simulink model "s_c_nbe_m1k"  (R2016b)
(part 4 of 198)

  [ct_sync] -> Subsystem10/5(in3)
  bus_create2/1(bus_out) -> [tvgtone_level0]
  bus_create3/1(bus_out) -> [tvgtone_level1]
  tvg_tone_levels/2(in_p0i) -> bus_create2/2(in2)
  tvg_tone_levels/3(in_p1r) -> bus_create3/1(in1)
  tvg_tone_levels/4(in_p1i) -> bus_create3/2(in2)
  tvg_tone_levels/1(in_p0r) -> bus_create2/1(in1)
  tvg_tone_targets/1(in_p0) -> Slice18/1
  tvg_tone_targets/2(in_p1) -> Slice19/1
  Constant51/1 -> tvg_tone_targets/1(sim_1)
  Constant52/1 -> tvg_tone_targets/2(sim_2)
  Constant37/1 -> tvg_tone_levels/4(sim_4)
  Constant2/1 -> tvg_tone_levels/1(sim_1)
  Constant27/1 -> tvg_tone_levels/3(sim_3)
  Constant5/1 -> tvg_tone_levels/2(sim_2)
  we_delay49/1(q) -> [ct_tag_insert_sel]
  edge_detect3/1 -> [ct_rst_err_latch]
  we_delay47/1(q) -> edge_detect3/1
  we_delay48/1(q) -> [ct_fake_data_error]
  we_delay13/1(q) -> [ct_tvg_en]
  we_delay50/1(q) -> [ct_tvg_en2]
  Constant7/1 -> ct_control0/5(sim_5)
  Constant21/1 -> ct_control0/4(sim_4)
  Constant20/1 -> ct_control0/3(sim_3)
  Constant22/1 -> ct_control0/2(sim_2)
  Constant15/1 -> ct_control0/1(sim_1)
  ct_control0/1(in_tvg_en) -> we_delay13/1(d)
  ct_control0/2(in_tvg_en2) -> we_delay50/1(d)
  ct_control0/3(in_rst_err_latch) -> we_delay47/1(d)
  ct_control0/4(in_fake_error) -> we_delay48/1(d)
  ct_control0/5(in_tag_insert) -> we_delay49/1(d)
  we_delay126/1(q) -> [obuf_read_gap]
  ct_control0/6(in_obuf_read_gap) -> we_delay126/1(d)
  Constant30/1 -> ct_control0/6(sim_6)
  we_delay41/1(q) -> [ct_num_xeng]
  we_delay112/1(q) -> [ct_num_xeng_recip]  "NUM_X_RECIP"
  ct_control1/2(in_num_x_recip) -> we_delay112/1(d)
  ct_control1/1(in_num_x) -> we_delay41/1(d)
  we_delay114/1(q) -> [ct_x_per_board]
  ct_control1/3(in_x_per_board) -> we_delay114/1(d)
  we_delay113/1(q) -> [ct_chans_per_board]
  ct_control2/1(in_chans_per_x) -> we_delay39/1(d)
  ct_control2/2(in_chans_per_board) -> we_delay113/1(d)
  we_delay115/1(q) -> [ct_x_per_board_recip]
  ct_control1/4(in_x_per_board_recip) -> we_delay115/1(d)
  we_delay38/1(q) -> [ct_num_x_boards]
  ct_control3/1(in_num_x_boards) -> we_delay38/1(d)
  we_delay37/1(q) -> [ct_num_x_boards_recip]
  ct_control3/2(in_num_x_boards_recip) -> we_delay37/1(d)
  Constant49/1 -> ct_control1/1(sim_1)
  Constant53/1 -> ct_control1/2(sim_2)
  Constant33/1 -> ct_control1/3(sim_3)
  Constant23/1 -> ct_control2/1(sim_1)
  Constant50/1 -> ct_control2/2(sim_2)
  Constant54/1 -> ct_control1/4(sim_4)
  Constant32/1 -> ct_control3/1(sim_1)
  Constant14/1 -> ct_control3/2(sim_2)
  Slice18/1 -> [tvgtone_p0]
  Slice19/1 -> [tvgtone_p1]
  Slice36/1 -> we_delay116/1(d)
  Constant38/1 -> ct_control4/1(sim_1)
  ct_control4/1(in_ct_board_offset) -> Slice36/1
  ct_control5/1(in_ct_freq_gen_offset) -> we_delay117/1(d)
  Constant39/1 -> ct_control5/1(sim_1)
  we_delay116/1(q) -> [ct_board_hmc_offset]
  we_delay117/1(q) -> [ct_freq_gen_offset]
  we_delay124/1(q) -> [ct_chans_per_x_recip]
  we_delay39/1(q) -> [ct_chans_per_x]  "PER_X"
  pipeline123/1(q) -> Counter13/1
  pipeline129/1(q) -> Counter13/2
  pipeline133/1(q) -> Counter11/1
  pipeline139/1(q) -> Counter11/2
  pipeline140/1(q) -> Counter15/1
  pipeline141/1(q) -> Counter15/2
  pipeline142/1(q) -> Counter7/1
  pipeline144/1(q) -> Counter7/2
  pipeline145/1(q) -> Counter6/2
  pipeline146/1(q) -> Counter6/1
  pipeline151/1(q) -> Counter9/2
  pipeline152/1(q) -> Counter9/1
  pipeline153/1(q) -> Counter8/2
  pipeline154/1(q) -> Counter8/1
  pipeline83/1(q) -> Counter14/1
  quant_snap_ctrl/1(in_single_channel) -> [quant_snap_single_channel]
  quant_snap_ctrl/2(in_channel_select) -> Slice3/1
  Subsystem6/1(out0) -> ct_dv_err/1(out_pktlen_err_cnt)
  Subsystem6/2(out1) -> ct_dv_err/2(out_dvblock_err_cnt)
  Subsystem8/1(Out1) -> ct_out_dv_rate/1(out_reg)
  Subsystem17/1(Out1) -> ct_in_dv_rate/1(out_reg)
  Subsystem10/1(out0) -> ct_sync_cnt/1(out_sync_in)
  Subsystem10/2(out1) -> ct_sync_cnt/2(out_rd_addr_arm_cnt)
  Subsystem10/3(out2) -> ct_sync_cnt/3(out_rd_sync_cnt)
  Subsystem10/4(out3) -> ct_sync_cnt/4(out_sync_out)
  Subsystem26/1(Out1) -> cd_out_dv_rate/1(out_reg)
  Subsystem25/1(Out1) -> cd_in_dv_rate/1(out_reg)
  phase1/1(in_initial) -> Reinterpret9/1
  phase1/2(in_delta) -> Reinterpret12/1
  delay_frac1/1(in_initial) -> Reinterpret5/1
  delay_whole1/1(in_initial) -> Reinterpret6/1
  Reinterpret5/1 -> Shift3/1
  Concat14/1 -> [ld_val1]
  Concat3/1 -> pipeline173/1(d)
  Concat9/1 -> pipeline174/1(d)
  Reinterpret10/1 -> Delay123/1
  Reinterpret11/1 -> Shift4/1
  delta_delay_frac1/1(in_initial) -> Reinterpret11/1
  delta_delay_whole1/1(in_initial) -> Reinterpret10/1
  Constant55/1 -> delay_whole1/1(sim_1)
  Constant62/1 -> delay_frac1/1(sim_1)
  Constant63/1 -> delta_delay_whole1/1(sim_1)
  Constant64/1 -> delta_delay_frac1/1(sim_1)
  Reinterpret12/1 -> Delay125/1
  Reinterpret9/1 -> Delay124/1
  Constant60/1 -> phase1/1(sim_1)
  Constant61/1 -> phase1/2(sim_2)
  Reinterpret6/1 -> Delay122/1
  Shift3/1 -> Concat3/2
  Shift4/1 -> Concat9/2
  Delay122/1 -> Concat3/1
  Delay123/1 -> Concat9/1
  Delay124/1 -> pipeline175/1(d)
  Delay125/1 -> pipeline176/1(d)
  pipeline173/1(q) -> Concat14/1
  pipeline174/1(q) -> Concat14/2
  pipeline175/1(q) -> Concat14/3
  pipeline176/1(q) -> Concat14/4
  [tl_cd1_load_time] -> tl_fd1/10(load_time)
  [tl_cd0_load_time] -> tl_fd0/10(load_time)
  Slice2/1 -> time_gen1/3(wr_val_in)
  pipeline209/1(q) -> time_gen/3(wr_val_in)
  [time80_48] -> Subsystem/1(time)
  Delay9/1 -> pipeline202/1(d), AddSub/1, Register1/1
  Delay11/1 -> pipeline203/1(d), AddSub/2, Register3/1
  From323/1 -> edge_detect11/1(in), pipeline205/1(d)
  edge_detect11/1(out) -> pipeline206/1(d)
  pipeline202/1(q) -> snap_time_check/1(in_time80_48)
  pipeline203/1(q) -> snap_time_check/2(in_pack_sync_time)
  pipeline204/1(q) -> snap_time_check/3(in_time_diff)
  pipeline205/1(q) -> snap_time_check/4(we)
  pipeline206/1(q) -> snap_time_check/5(trig)
  pipeline211/1(q) -> dds_fft_phase_offset/1(out_offset)
  From325/1 -> pipeline213/1(d)
  pipeline213/1(q) -> snap_adc0/10(in_sync)
  [time80] -> pipeline209/1(d)
  [d80_adc0] -> bus_expand9/1(bus_in)
  bus_expand9/4(out5) -> pipeline193/1(d)
  bus_expand9/5(out4) -> pipeline192/1(d)
  bus_expand9/1(msb_out8) -> pipeline196/1(d)
  bus_expand9/2(out7) -> pipeline195/1(d)
  bus_expand9/3(out6) -> pipeline194/1(d)
  bus_expand9/6(out3) -> pipeline191/1(d)
  bus_expand9/7(out2) -> pipeline190/1(d)
  bus_expand9/8(lsb_out1) -> pipeline189/1(d)
  [valid80] -> pipeline182/1(d), pipeline188/1(d)
  [cnt_rst] -> pipeline226/1(d)
  pipeline225/1(q) -> Counter10/2
  pipeline226/1(q) -> Counter10/1
  [pfb_sync] -> Logical16/1
  Logical16/1 -> pipeline225/1(d)
  [pfb_dv] -> Logical16/2
  [cnt_rst] -> pipeline230/1(d)
  pipeline229/1(q) -> Counter12/2
  pipeline230/1(q) -> Counter12/1
  [ddc_sync] -> Logical17/1
  [ddc_dvalid] -> Logical17/2
  Logical17/1 -> pipeline229/1(d)
  [sys_rst] -> pipeline232/1(d)
  pipeline232/1(q) -> Counter16/1
  pipeline233/1(q) -> Counter16/2
  [valid80] -> Logical18/2
  [sync80] -> Logical18/1
  Logical18/1 -> pipeline233/1(d)
  nb_pfb/3(pol0_out) -> Delay130/1
  nb_pfb/4(pol1_out) -> Delay131/1
  [ddc_pol0] -> nb_pfb/2(pol0)
  [ddc_pol1] -> nb_pfb/3(pol1)
  [ddc_dvalid] -> nb_pfb/4(dvalid)
  fft_shift/1(in_fft_shift) -> fft_shift_munge/1(din)
  pipeline85/1(q) -> [fft_shift]
  Constant67/1 -> fft_shift/1(sim_1)
  [fft_shift] -> nb_pfb/5(fft_shift)
  Delay127/1 -> [pfb_sync]
  phase0/1(in_initial) -> Reinterpret2/1
  phase0/2(in_delta) -> Reinterpret3/1
  delay_frac0/1(in_initial) -> Reinterpret18/1
  delay_whole0/1(in_initial) -> Reinterpret19/1
  Reinterpret18/1 -> Shift1/1
  Concat11/1 -> pipeline169/1(d)
  Concat12/1 -> pipeline170/1(d)
  Reinterpret20/1 -> Delay119/1
  Reinterpret21/1 -> Shift2/1
  delta_delay_frac0/1(in_initial) -> Reinterpret21/1
  delta_delay_whole0/1(in_initial) -> Reinterpret20/1
  Constant10/1 -> delay_whole0/1(sim_1)
  Constant76/1 -> delay_frac0/1(sim_1)
  Constant77/1 -> delta_delay_whole0/1(sim_1)
  Constant78/1 -> delta_delay_frac0/1(sim_1)
  Reinterpret3/1 -> Delay121/1
  Reinterpret2/1 -> Delay120/1
  Constant12/1 -> phase0/1(sim_1)
  Constant75/1 -> phase0/2(sim_2)
  Reinterpret19/1 -> Delay118/1
  Shift1/1 -> Concat11/2
  Shift2/1 -> Concat12/2
  Delay118/1 -> Concat11/1
  Delay119/1 -> Concat12/1
  Delay120/1 -> pipeline171/1(d)
  Delay121/1 -> pipeline172/1(d)
  pipeline169/1(q) -> Concat22/1
  pipeline170/1(q) -> Concat22/2
  pipeline171/1(q) -> Concat22/3
  pipeline172/1(q) -> Concat22/4
  Concat22/1 -> [ld_val0]
  Counter15/1 -> pipeline94/1(d)
  Counter6/1 -> pipeline95/1(d)
  Counter12/1 -> pipeline109/1(d)
  Counter7/1 -> pipeline117/1(d)
  Counter10/1 -> pipeline119/1(d)
  Counter8/1 -> pipeline118/1(d)
  Counter9/1 -> pipeline159/1(d)
  Counter13/1 -> pipeline4/1(d)
  Counter16/1 -> pipeline86/1(d)
  Counter11/1 -> pipeline87/1(d)
  pipeline4/1(q) -> cd_status/1(out_sync80)
  pipeline86/1(q) -> cd_status/2(out_sync80_1)
  pipeline87/1(q) -> cd_status/3(out_hmc_sync_out)
  pipeline94/1(q) -> ddc_status/1(out_in_sync_cnt)
  pipeline95/1(q) -> ddc_status/2(out_out_sync_cnt)
  pipeline109/1(q) -> ddc_status/3(out_out_sync_cnt1)
  pipeline117/1(q) -> ddc_status/4(out_dv_cnt)
  pipeline118/1(q) -> nb_status/1(out_out_sync_cnt)
  pipeline119/1(q) -> nb_status/2(out_out_sync_cnt1)
  pipeline159/1(q) -> nb_status/3(out_dv_cnt)
  [tg_pfb_sync] -> pipeline238/1(d)
  [cnt_rst] -> pipeline239/1(d)
  pipeline239/1(q) -> Counter17/1
  [fdfs_sync] -> pipeline240/1(d)
  [cnt_rst] -> pipeline241/1(d)
  pipeline241/1(q) -> Counter18/1
  Counter18/1 -> pipeline177/1(d)
  Counter17/1 -> pipeline168/1(d)
  pipeline168/1(q) -> fdfs_sync_cnt/1(out_pfb_sync_cnt)
  pipeline177/1(q) -> fdfs_sync_cnt/2(out_fdfs_sync_cnt)
  pipeline178/1(q) -> quant_sync_cnt/1(out_reg)
  tl_fd1/3(sync_out) -> phase_compensation1/1(sync_in)
  tl_fd1/4(dout) -> phase_compensation1/2(din)
  tl_fd1/5(dvalid) -> phase_compensation1/3(en)
  tl_fd1/2(enable) -> phase_compensation1/5(load_value)
  tl_fd1/1(value) -> phase_compensation1/4(delay_value)
  From241/1 -> Delay96/1
  From74/1 -> Delay97/1
  calc_adc_sum_sq0/1(mean_pwr) -> Delay94/1
  Delay94/1 -> adc_pwr0/1(out_reg)
  Delay95/1 -> adc_pwr1/1(out_reg)
  Delay96/1 -> calc_adc_sum_sq0/1(adc_in)
  Delay97/1 -> calc_adc_sum_sq1/1(adc_in)
  calc_adc_sum_sq1/1(mean_pwr) -> Delay95/1
  Delay102/1 -> adc_dev0/1(out_max)
  Delay101/1 -> adc_dev0/2(out_min)
  calc_adc_sum_sq0/2(max) -> Delay102/1
  calc_adc_sum_sq0/3(min) -> Delay101/1
  Delay104/1 -> adc_dev1/1(out_max)
  Delay103/1 -> adc_dev1/2(out_min)
  calc_adc_sum_sq1/2(max) -> Delay104/1
  calc_adc_sum_sq1/3(min) -> Delay103/1
  Delay112/1 -> calc_pfb_pwr0/1(adc_in)
  [pfb_d144_0] -> Delay112/1
  Delay107/1 -> calc_pfb_pwr1/1(adc_in)
  [pfb_d144_1] -> Delay107/1
  calc_pfb_pwr0/1(mean_pwr) -> pfb_pwr0/1(out_scale8)
  [pfb_dv] -> Delay106/1
  Delay106/1 -> calc_pfb_pwr0/2(valid_in)
  [pfb_dv] -> Delay110/1
  Delay110/1 -> calc_pfb_pwr1/2(valid_in)
  calc_pfb_pwr1/1(mean_pwr) -> pfb_pwr1/1(out_scale8)
  [q_d64_0] -> Delay116/1
  [q_d64_1] -> Delay117/1
  calc_quant_pwr0/1(mean_pwr) -> pipeline160/1(d)
  calc_quant_pwr1/1(mean_pwr) -> pipeline165/1(d)
  Delay116/1 -> calc_quant_pwr0/1(adc_in)
  Delay117/1 -> calc_quant_pwr1/1(adc_in)
  pipeline160/1(q) -> quant_pwr0/1(out_reg)
  pipeline165/1(q) -> quant_pwr1/1(out_reg)
  [q_dv] -> Delay114/1
  Delay114/1 -> calc_quant_pwr0/2(valid_in)
  [q_dv] -> Delay115/1
  Delay115/1 -> calc_quant_pwr1/2(valid_in)
  bus_expand8/2(lsb_out1) -> pipeline211/1(d)
  bus_expand8/1(msb_out2) -> pipeline179/1(d)
  pipeline179/1(q) -> dds_fft_bin/1(out_bin)
  [dds_fft_phase_offset] -> bus_expand8/1(bus_in)
  Constant65/1 -> ts_ss_lock/1(sim_1)
  ts_ss_lock/1(in_en) -> pipeline180/1(d)
  pipeline180/1(q) -> [ts_ss_lock]
  [ts_ss_lock] -> Mux7/1
  Mux7/1 -> edge_detect13/1(in)
  arm_ts_ss_lock/1(in_en) -> pipeline181/1(d)
  pipeline181/1(q) -> edge_detect12/1(in)
  Constant69/1 -> arm_ts_ss_lock/1(sim_1)
  edge_detect12/1(out) -> [arm_ts_ss_lock]
  [sync80] -> Mux7/2, pipeline187/1(d)
  [arm_ts_ss_rst] -> ss_time_trig_adc/2(rst)
  [arm_ts_ss_lock] -> ss_time_trig_adc/3(arm)
  ss_time_trig_adc/1(trig) -> Mux7/3
  edge_detect13/1(out) -> pipeline198/1(d), pipeline186/1(d)
  Constant70/1 -> ss_trig_time_in_lsw/1(sim_1)
  ss_trig_time_in_lsw/1(in_time) -> pipeline183/1(d)
  [ss_trig_time_in] -> ss_time_trig_adc/4(trig_time_in)
  ss_time_trig_adc/2(trig_time) -> Slice6/1
  [ts_ss_lock] -> Mux8/1
  Mux8/1 -> edge_detect14/1(in)
  ss_time_trig_quant/1(trig) -> Mux8/3
  quant_snap_filter0/3(packet_sync_out) -> Mux8/2
  edge_detect14/1(out) -> pipeline199/1(d), pipeline197/1(d)
  ss_time_trig_quant/2(trig_time) -> pipeline200/1(d)
  arm_ss_ts_rst/1(in_rst) -> pipeline184/1(d)
  pipeline184/1(q) -> edge_detect15/1(in)
  Constant68/1 -> arm_ss_ts_rst/1(sim_1)
  edge_detect15/1(out) -> [arm_ts_ss_rst]
  pipeline185/1(q) -> snap_adc/12(in_trig_time)
  pipeline186/1(q) -> snap_adc/11(in_trig)
  pipeline187/1(q) -> snap_adc/10(in_sync)
  pipeline188/1(q) -> snap_adc/9(in_dv)
  pipeline190/1(q) -> snap_adc/7(in_p0_d6)
  pipeline191/1(q) -> snap_adc/6(in_p0_d5)
  pipeline192/1(q) -> snap_adc/5(in_p0_d4)
  pipeline189/1(q) -> snap_adc/8(in_p0_d7)
  pipeline194/1(q) -> snap_adc/3(in_p0_d2)
  pipeline195/1(q) -> snap_adc/2(in_p0_d1)
  pipeline193/1(q) -> snap_adc/4(in_p0_d3)
  pipeline196/1(q) -> snap_adc/1(in_p0_d0)
  pipeline197/1(q) -> snap_quant0/9(in_trig)
  pipeline200/1(q) -> snap_quant0/10(in_trig_time)
  pipeline214/1(q) -> snap_quant0/8(in_imag3)
  pipeline201/1(q) -> snap_quant0/7(in_real3)
  pipeline217/1(q) -> snap_quant0/6(in_imag2)
  pipeline215/1(q) -> snap_quant0/5(in_real2)
  pipeline218/1(q) -> snap_quant0/3(in_real1)
  pipeline219/1(q) -> snap_quant0/4(in_imag1)
  pipeline220/1(q) -> snap_quant0/1(in_real0)
  pipeline221/1(q) -> snap_quant0/2(in_imag0)
  pipeline222/1(q) -> snap_quant0/11(we)
  [time80_48] -> ss_time_trig_adc/1(current_time)
  [arm_ts_ss_rst] -> ss_time_trig_quant/2(rst)
  [arm_ts_ss_lock] -> ss_time_trig_quant/3(arm)
  [ss_trig_time_in] -> ss_time_trig_quant/4(trig_time_in)
  [time80_48] -> ss_time_trig_quant/1(current_time)
  Slice6/1 -> pipeline185/1(d)
  ss_trig_time_in_msw/1(in_time) -> pipeline224/1(d)
  Constant71/1 -> ss_trig_time_in_msw/1(sim_1)
  pipeline224/1(q) -> Concat/1
  pipeline183/1(q) -> Concat/2
  Concat/1 -> [ss_trig_time_in]
  pipeline240/1(q) -> Logical19/1
  Logical19/1 -> Counter18/2
  pipeline238/1(q) -> Logical20/1
  Logical20/1 -> Counter17/2
  [fdfs_dv] -> pipeline227/1(d)
  pipeline227/1(q) -> Logical19/2
  [tg_pfb_dv] -> pipeline235/1(d)
  pipeline235/1(q) -> Logical20/2
  pipeline158/1(q) -> Logical21/1
  Logical21/1 -> Counter14/2
  pipeline236/1(q) -> Logical21/2
  [q_dv] -> pipeline236/1(d)
  [pfbin_d0] -> bus_expand10/1(bus_in)
  [pfbin_dv] -> pipeline237/1(d), pipeline245/1(d)
  [ts_ss_lock] -> Mux9/1
  Mux9/1 -> edge_detect16/1(in)
  [pfbin_sync] -> Mux9/2, pipeline244/1(d)
  [arm_ts_ss_rst] -> ss_time_trig_pfbin/2(rst)
  [arm_ts_ss_lock] -> ss_time_trig_pfbin/3(arm)
  ss_time_trig_pfbin/1(trig) -> Mux9/3
  edge_detect16/1(out) -> pipeline46/1(d), pipeline243/1(d)
  [ss_trig_time_in] -> ss_time_trig_pfbin/4(trig_time_in)
  ss_time_trig_pfbin/2(trig_time) -> Slice23/1
  pipeline242/1(q) -> snap_pfbin/12(in_trig_time)
  pipeline243/1(q) -> snap_pfbin/11(in_trig)
  pipeline244/1(q) -> snap_pfbin/10(in_sync)
  pipeline245/1(q) -> snap_pfbin/9(in_dv)
  pipeline247/1(q) -> snap_pfbin/7(in_p0_d6)
  pipeline248/1(q) -> snap_pfbin/6(in_p0_d5)
  pipeline249/1(q) -> snap_pfbin/5(in_p0_d4)
  pipeline246/1(q) -> snap_pfbin/8(in_p0_d7)
  pipeline251/1(q) -> snap_pfbin/3(in_p0_d2)
  pipeline252/1(q) -> snap_pfbin/2(in_p0_d1)
  pipeline250/1(q) -> snap_pfbin/4(in_p0_d3)
  pipeline253/1(q) -> snap_pfbin/1(in_p0_d0)
  [time80_48] -> ss_time_trig_pfbin/1(current_time)
  Slice23/1 -> pipeline242/1(d)
  pipeline237/1(q) -> snap_pfbin/13(we)
  Delay130/1 -> [pfb_d144_0]
  Delay131/1 -> [pfb_d144_1]
  Delay128/1 -> [pfb_dv]
  pipeline182/1(q) -> snap_adc/13(we)
  pipeline198/1(q) -> snap_adc/14(trig)
  pipeline46/1(q) -> snap_pfbin/14(trig)
  pipeline199/1(q) -> snap_quant0/12(trig)
  complexify/1(Out1) -> Delay111/1
  complexify1/1(Out1) -> Delay113/1
  cwg_cos/3(rpt_rst) -> Terminator65/1
  cwg_cos/2(dvalid) -> Terminator14/1
  Constant74/1 -> freq_cwg_osc/1(sim_1)
  [sys_relock] -> cwg_cos/3(rst)
  Constant72/1 -> cwg_cos/2(scale)
  Constant79/1 -> cwg_cos/4(repeat_en)
  Constant81/1 -> cwg_cos/5(repeat_length)
  [tg_dds_dvalid] -> cwg_cos/6(en)
  cwg_cos/1(bus_out) -> [osc_cos_ddc0]
  [ddc_freq] -> dds_freq_idx_offset_calc/1(ddc_freq)
  dds_freq_idx_offset_calc/1(dds_fftbin_offset) -> [dds_fft_phase_offset]
  [osc_freq] -> [ddc_freq], cwg_cos/1(freq)
  [tg_dds_dvalid] -> cwg_sin/6(en)
  Constant80/1 -> cwg_sin/4(repeat_en)
  Constant57/1 -> cwg_sin/2(scale)
  Constant82/1 -> cwg_sin/5(repeat_length)
  freq_cwg_osc/1(in_frequency) -> [osc_freq]
  [sys_relock] -> cwg_sin/3(rst)
  [osc_freq] -> cwg_sin/1(freq)
  cwg_sin/2(dvalid) -> Terminator2/1
  cwg_sin/3(rpt_rst) -> Terminator4/1
  cwg_sin/1(bus_out) -> [osc_sin_ddc0]
  [osc_cos_ddc0] -> re_im_interleave/1(In1)
  [osc_sin_ddc0] -> re_im_interleave/2(In2)
  re_im_interleave/1(Out1) -> [osc_cmplx]
  Delay108/1 -> Delay126/1
  Delay109/1 -> [ddc_sync_in]
  [osc_cos_ddc0] -> bus_expand11/1(bus_in)
  bus_expand11/4(out5) -> pipeline261/1(d)
  bus_expand11/5(out4) -> pipeline260/1(d)
  bus_expand11/1(msb_out8) -> pipeline264/1(d)
  bus_expand11/2(out7) -> pipeline263/1(d)
  bus_expand11/3(out6) -> pipeline262/1(d)
  bus_expand11/6(out3) -> pipeline259/1(d)
  bus_expand11/7(out2) -> pipeline258/1(d)
  bus_expand11/8(lsb_out1) -> pipeline257/1(d)
  [ddc_dv_in] -> pipeline256/1(d), pipeline216/1(d)
  [ts_ss_lock] -> Mux10/1
  Mux10/1 -> edge_detect18/1(in)
  [ddc_sync_in] -> Mux10/2, pipeline255/1(d)
  [arm_ts_ss_rst] -> ss_time_trig_pfbin1/2(rst)
  [arm_ts_ss_lock] -> ss_time_trig_pfbin1/3(arm)
  ss_time_trig_pfbin1/1(trig) -> Mux10/3
  edge_detect18/1(out) -> pipeline254/1(d), pipeline265/1(d)
  [ss_trig_time_in] -> ss_time_trig_pfbin1/4(trig_time_in)
  ss_time_trig_pfbin1/2(trig_time) -> Slice24/1
  pipeline223/1(q) -> snap_cos/12(in_trig_time)
  pipeline254/1(q) -> snap_cos/11(in_trig)
  pipeline255/1(q) -> snap_cos/10(in_sync)
  pipeline256/1(q) -> snap_cos/9(in_dv)
  pipeline258/1(q) -> snap_cos/7(in_p0_d6)
  pipeline259/1(q) -> snap_cos/6(in_p0_d5)
  pipeline260/1(q) -> snap_cos/5(in_p0_d4)
  pipeline257/1(q) -> snap_cos/8(in_p0_d7)
  pipeline262/1(q) -> snap_cos/3(in_p0_d2)
  pipeline263/1(q) -> snap_cos/2(in_p0_d1)
  pipeline261/1(q) -> snap_cos/4(in_p0_d3)
  pipeline264/1(q) -> snap_cos/1(in_p0_d0)
  [time80_48] -> ss_time_trig_pfbin1/1(current_time)
  Slice24/1 -> pipeline223/1(d)
  pipeline216/1(q) -> snap_cos/13(we)
  pipeline265/1(q) -> snap_cos/14(trig)
  Delay126/1 -> [ddc_dv_in]
  Delay129/1 -> [ddc_pol0_in]
  Delay132/1 -> [ddc_pol1_in]
  bus_expand10/8(lsb_out1) -> pipeline246/1(d)
  bus_expand10/7(out2) -> pipeline247/1(d)
  bus_expand10/6(out3) -> pipeline248/1(d)
  bus_expand10/5(out4) -> pipeline249/1(d)
  bus_expand10/4(out5) -> pipeline250/1(d)
  bus_expand10/3(out6) -> pipeline251/1(d)
  bus_expand10/2(out7) -> pipeline252/1(d)
  bus_expand10/1(msb_out8) -> pipeline253/1(d)
  pipeline267/1(q) -> ddc_status1/2(out_ddc_of1)
  pipeline266/1(q) -> ddc_status1/1(out_ddc_of0)
  Counter19/1 -> pipeline266/1(d)
  Counter20/1 -> pipeline267/1(d)
  [cnt_rst] -> pipeline268/1(d)
  pipeline269/1(q) -> Counter19/2
  pipeline268/1(q) -> Counter19/1
  pipeline271/1(q) -> Counter20/2
  pipeline270/1(q) -> Counter20/1
  [cnt_rst] -> pipeline270/1(d)
  DDC/5(ddc_of) -> [ddc_of]
  [ddc_of] -> bus_expand12/1(bus_in)
  bus_expand12/1(msb_out2) -> pipeline269/1(d)
  bus_expand12/2(lsb_out1) -> pipeline271/1(d)
  Concat16/1 -> time_gen_dds/6(rd_misc_in)
  time_gen_dds/4(rd_misc_out) -> bus_expand13/1(bus_in)
  [sync_tl_cd0] -> time_gen_dds/1(wr_sync_in)
  [dvalid_tl_cd0] -> time_gen_dds/2(wr_en)
  [pfbin_sync] -> time_gen_dds/4(rd_sync_in)
  [pfbin_dv] -> time_gen_dds/5(rd_en)
  time_gen_dds/1(rd_sync_out) -> [tg_dds_sync]
  time_gen_dds/2(rd_dvalid) -> [tg_dds_dvalid]
  time_gen_dds/3(rd_val_out) -> [tg_dds_time_out]
  [pfbin_d0] -> Concat16/1
  [pfbin_d1] -> Concat16/2
  bus_expand13/1(msb_out2) -> [tg_dds_data_p0]
  bus_expand13/2(lsb_out1) -> [tg_dds_data_p1]
  [tg_dds_time_out] -> cwg_sin/7(time_in)
  [tg_dds_time_out] -> cwg_cos/7(time_in)
  [time80_tl_cd0] -> time_gen_dds/3(wr_val_in)
  pipeline82/1(q) -> snap_dds_tg/2(in_sync)
  pipeline272/1(q) -> snap_dds_tg/3(in_dv)
  pipeline49/1(q) -> snap_dds_tg/4(we)
  pipeline281/1(q) -> snap_dds_tg/5(trig)
  pipeline50/1(q) -> snap_dds_tg/1(in_time_slice)
  [tg_dds_sync] -> pipeline82/1(d), pipeline281/1(d)
  [tg_dds_dvalid] -> pipeline272/1(d), pipeline49/1(d)
  [tg_dds_time_out] -> Slice/1
  Slice/1 -> pipeline50/1(d)
  fft_shift_munge/1(dout) -> pipeline85/1(d)
  Constant44/1 -> ct_control0/7(sim_7)
  nb_pfb/5(pfb_of) -> Delay133/1
  Delay133/1 -> [pfb_of]
  Constant13/1 -> ct_control3/3(sim_3)
  ct_control3/3(in_chans_per_x_recip) -> we_delay124/1(d)
